simulink model "ssc_hydraulic_lift"  (R2025a)
settings: Solver=ode23t  StartTime=0.0  StopTime=20  MaxStep=0.02  RelTol=1e-3  AbsTol=1e-4  EnableMultiTasking=on
PreLoadFcn:
  | warning('off','Simulink:Commands:LoadMdlParameterizedLink');
PostLoadFcn:
  | warning off sm:compiler:topologyAnalysis:DanglingBlock
  | warning off Simulink:SL_SolverMaskedZC;
  | warning off Simulink:SL_SolverIgnoredZCBracketing;
  | warning off Simulink:Engine:SolverMinStepNonlinearIterWarnForDAE;
  | warning off simscape:compiler:sli:init:SolverNotRecommended
  | warning off Simulink:Engine:UsingDiscreteSolver
  | warning('off','sm:sli:setup:compile:LocalSolverNotSupported')
  | warning off physmod:simscape:compiler:sli:init:SolverNotRecommended
  | warning off sm:sli:visualization:ModelRefNotSupported
  | warning off Simulink:modelReference:ProtectedModelCallbackLostWarning
StartFcn:
  | tic;
StopFcn:
  | Elapsed_Sim_Time = toc;
  | disp(['Elapsed Sim Time = ' num2str(Elapsed_Sim_Time)]);
undefined symbols (not defined in the file): actuator_hs_b, actuator_hs_k, Local, motor_damping, Scissor_Lift_Param, sigbuilder_block, X, Y, Z
libraries: fl_lib x108, sm_lib x41, Scissor_Parts_Lib x24, nesl_utility x6, SimscapeFluids_lib x2, Custom_lib x2, slpidlib x1, fl_ps_legacy_lib x1, ee_lib x1, Motor_Lib x1, sdl_lib x1
(part 2 of 3)

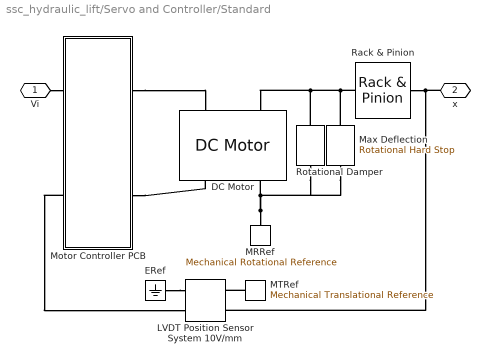
== system ssc_hydraulic_lift/Servo and Controller/Standard ==
  DC Motor : ee_lib/Electromechanical/Brushed Motors/DC Motor  field_option=ee.enum.field_option.pm  Rf=100 Ohm  Lf=1 H  Laf=0.15 H  If0=0 A  parameterization=1  Ra=R Ohm  La=L H  emf_or_torque=1  Kv=Kt V/(rad/s)  Ki=6.876e-4 N*m/A  T_stall=2.4e-4 N*m  w_max=1.91e+4 rpm  w_rated=1.5e+4 rpm  P_rated=0.08 W  V_rated=1.5 V  lam_param=1  i_noload=0 A  V_i_noload=1.5 V  J=J kg*m^2  lam=0 N*m/(rad/s)  speed0=0 rpm  alpha=3.93e-3 1/K  Tmeas=25 degC  thermal_mass=100 J/K  initial_temperature=25 degC
  ERef : fl_lib/Electrical/Electrical Elements/Electrical Reference
  LVDT Position Sensor System 10V/mm : Motor_Lib/Custom/LVDT Position Sensor System 10V//mm  SystemSampleTime=-1  VariantActivationTime=update diagram  EmptyChoice=off  PassThrough=off  PassThroughVariantControl=(default)  EmptyChoiceVariantControl=(default)  AllowFlexibleInterface=on  Latency=0  AutoFrameSizeCalculation=off
  MRRef : fl_lib/Mechanical/Rotational Elements/Mechanical Rotational Reference
  MTRef : fl_lib/Mechanical/Translational Elements/Mechanical Translational Reference
  Max Deflection : fl_lib/Mechanical/Rotational Elements/Rotational Hard Stop  upper_bnd=x_max*1e-3/G rad  lower_bnd=-x_max*1e-3/G rad  model=3  stiff_up=1e+06 N*m/rad  stiff_low=1e+06 N*m/rad  D_up=0.05 N*m/(rad/s)  D_low=0.05 N*m/(rad/s)  transition=0.001 rad  coeff_rest=0.7  w_tol=0.1 rad/s  trq_tol=0.001 N*m  w_specify=off  w_priority=None  w=0 rad/s  w_nominal_specify=off  w_nominal_value=1  w_nominal_unit=rad/s  t_specify=off  t_priority=None  t=0 N*m  t_nominal_specify=off  t_nominal_value=1  t_nominal_unit=N*m  phi_specify=on  phi_priority=High  phi=0 rad  phi_nominal_specify=off  phi_nominal_value=1  phi_nominal_unit=rad  M_specify=off  M_priority=None  M=0
  Motor Controller PCB : Subsystem
  Rack & Pinion : sdl_lib/Gears/Rotational- Translational/Rack & Pinion  param=1  radius=G m  n_teeth=20  x_tooth=5 mm  rack_direction_sign=1  friction_model=1  efficiency=0.8  temperature_TLU=[ 280 300 320 ] K  efficiency_TLU=[ 0.95 0.9 0.85 ]  pwr_thr=0.001 W  mu_visc_P=0 N*m/(rad/s)  mu_visc_R=0 N/(m/s)  thermal_mass=50 J/K  temperature_specify=off  temperature_priority=High  temperature=300 K  temperature_nominal_specify=off  temperature_nominal_value=1  temperature_nominal_unit=K
      settings: InternalSimscapePortConfiguration="{\"Bottom\":[],\"Left\":[{\"id\":\"P\",\"label\":\"P\",\"type\":\"foundation.mechanical.rotational.rotational\"}],\"Right\":[{\"id\":\"R\",\"label\":\"R\",\"type\":\"foundation.mechanical.translational.translational\"}],\"Top\":[]}"
  Rotational Damper : fl_lib/Mechanical/Rotational Elements/Rotational Damper  D=lambda N*m/(rad/s)  w_specify=off  w_priority=None  w=0 rad/s  w_nominal_specify=off  w_nominal_value=1  w_nominal_unit=rad/s  t_specify=off  t_priority=None  t=0 N*m  t_nominal_specify=off  t_nominal_value=1  t_nominal_unit=N*m
  Vi : PMIOPort  Side=Left
  x : PMIOPort  Port=2  Side=Right
  connections:
  Rack & Pinion/RConn1 -- LVDT Position Sensor System 10V/mm/LConn2 -- x/RConn1
  MTRef/LConn1 -- LVDT Position Sensor System 10V/mm/LConn1
  Motor Controller PCB/LConn2 -- LVDT Position Sensor System 10V/mm/RConn2
  ERef/LConn1 -- LVDT Position Sensor System 10V/mm/RConn1
  Motor Controller PCB/RConn2 -- DC Motor/RConn1
  Rack & Pinion/LConn1 -- DC Motor/LConn2 -- Rotational Damper/LConn1 -- Max Deflection/LConn1
  MRRef/LConn1 -- Max Deflection/RConn1 -- Rotational Damper/RConn1 -- DC Motor/RConn2
  Motor Controller PCB/RConn1 -- DC Motor/LConn1
  Vi/RConn1 -- Motor Controller PCB/LConn1

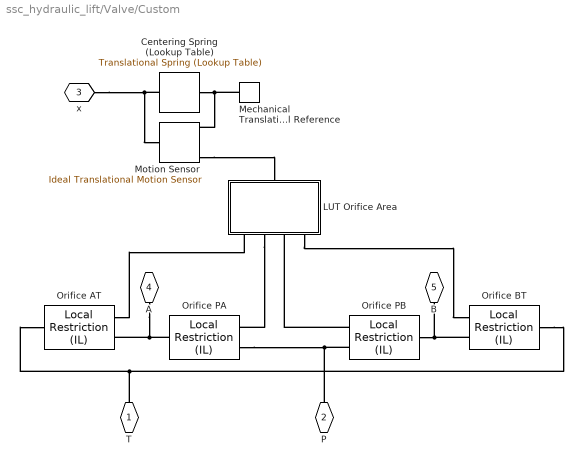
== system ssc_hydraulic_lift/Valve/Custom ==
  Centering Spring (Lookup Table) : Custom_lib/Mechanical/Translational Spring (Lookup Table)  xd=[-1 -0.9 0,0.9 1]*x_max mm  kd=[100,10,10,10,100] N/m  f_specify=off  f_priority=High  f=0 N  f_nominal_specify=off  f_nominal_value=1  f_nominal_unit=N  x_specify=off  x_priority=High  x=0 m  x_nominal_specify=off  x_nominal_value=1  x_nominal_unit=m  v_specify=off  v_priority=High  v=0 m/s  v_nominal_specify=off  v_nominal_value=1  v_nominal_unit=m/s  k_specify=off  k_priority=High  k=0 N/m  k_nominal_specify=off  k_nominal_value=1  k_nominal_unit=N/m
      settings: InternalSimscapePortConfiguration="{\"Bottom\":[],\"Left\":[{\"id\":\"c\",\"label\":\"c\",\"type\":\"foundation.mechanical.translational.translational\"}],\"Right\":[{\"id\":\"r\",\"label\":\"r\",\"type\":\"foundation.mechanical.translational.translational\"}],\"Top\":[]}"
  LUT Orifice Area : Subsystem
  Mechanical Translational Reference : fl_lib/Mechanical/Translational Elements/Mechanical Translational Reference
  Motion Sensor : fl_lib/Mechanical/Mechanical Sensors/Ideal Translational Motion Sensor  reference=foundation.enum.MeasurementReference.difference  acceleration_port=false  velocity_port=true  position_port=true  offset=0 m
  Orifice AT : fl_lib/Isothermal Liquid/Elements/Local Restriction (IL)  restriction_type=foundation.enum.restriction_type.variable  restriction_area=1e-3 m^2  min_area=1e-12 m^2  max_area=1e10 m^2  area=inf m^2  Cd=K_V  Re_c=12  pressure_recovery=false
      settings: LibrarySourceBlock=fl_lib/Isothermal Liquid/Elements/Local Restriction (IL)  InternalSimscapePortConfiguration="{\"Bottom\":[],\"Left\":[{\"id\":\"A\",\"label\":\"A\",\"type\":\"foundation.isothermal_liquid.isothermal_liquid\"},{\"id\":\"AR\",\"label\":\"AR\",\"type\":\"input\"}],\"Right\":[{\"id\":\"B\",\"label\":\"B\",\"type\":\"foundation.isothermal_liquid.isothermal_liquid\"}],\"Top\":[]}"
  Orifice BT : fl_lib/Isothermal Liquid/Elements/Local Restriction (IL)  restriction_type=foundation.enum.restriction_type.variable  restriction_area=1e-3 m^2  min_area=1e-12 m^2  max_area=1e10 m^2  area=inf m^2  Cd=K_V  Re_c=12  pressure_recovery=false
      settings: LibrarySourceBlock=fl_lib/Isothermal Liquid/Elements/Local Restriction (IL)  InternalSimscapePortConfiguration="{\"Bottom\":[],\"Left\":[{\"id\":\"A\",\"label\":\"A\",\"type\":\"foundation.isothermal_liquid.isothermal_liquid\"},{\"id\":\"AR\",\"label\":\"AR\",\"type\":\"input\"}],\"Right\":[{\"id\":\"B\",\"label\":\"B\",\"type\":\"foundation.isothermal_liquid.isothermal_liquid\"}],\"Top\":[]}"
  Orifice PA : fl_lib/Isothermal Liquid/Elements/Local Restriction (IL)  restriction_type=foundation.enum.restriction_type.variable  restriction_area=1e-3 m^2  min_area=1e-12 m^2  max_area=1e10 m^2  area=inf m^2  Cd=K_V  Re_c=12  pressure_recovery=false
      settings: LibrarySourceBlock=fl_lib/Isothermal Liquid/Elements/Local Restriction (IL)  InternalSimscapePortConfiguration="{\"Bottom\":[],\"Left\":[{\"id\":\"A\",\"label\":\"A\",\"type\":\"foundation.isothermal_liquid.isothermal_liquid\"},{\"id\":\"AR\",\"label\":\"AR\",\"type\":\"input\"}],\"Right\":[{\"id\":\"B\",\"label\":\"B\",\"type\":\"foundation.isothermal_liquid.isothermal_liquid\"}],\"Top\":[]}"
  Orifice PB : fl_lib/Isothermal Liquid/Elements/Local Restriction (IL)  restriction_type=foundation.enum.restriction_type.variable  restriction_area=1e-3 m^2  min_area=1e-12 m^2  max_area=1e10 m^2  area=inf m^2  Cd=K_V  Re_c=12  pressure_recovery=false
      settings: LibrarySourceBlock=fl_lib/Isothermal Liquid/Elements/Local Restriction (IL)  InternalSimscapePortConfiguration="{\"Bottom\":[],\"Left\":[{\"id\":\"A\",\"label\":\"A\",\"type\":\"foundation.isothermal_liquid.isothermal_liquid\"},{\"id\":\"AR\",\"label\":\"AR\",\"type\":\"input\"}],\"Right\":[{\"id\":\"B\",\"label\":\"B\",\"type\":\"foundation.isothermal_liquid.isothermal_liquid\"}],\"Top\":[]}"
  T : PMIOPort  Tag=PMCPort  Side=Left
  P : PMIOPort  Tag=PMCPort  Port=2  Side=Left
  x : PMIOPort  Tag=PMCPort  Port=3  Side=Left
  A : PMIOPort  Tag=PMCPort  Port=4  Side=Right
  B : PMIOPort  Tag=PMCPort  Port=5  Side=Right
  connections:
  P/RConn1 -- Orifice PB/LConn1 -- Orifice PA/LConn1
  Mechanical Translational Reference/LConn1 -- Centering Spring (Lookup Table)/RConn1 -- Motion Sensor/RConn1
  x/RConn1 -- Centering Spring (Lookup Table)/LConn1 -- Motion Sensor/LConn1
  Motion Sensor/RConn3 -- LUT Orifice Area/LConn1
  Orifice AT/LConn2 -- LUT Orifice Area/RConn1
  Orifice PB/RConn1 -- Orifice BT/LConn1 -- B/RConn1
  Orifice PB/LConn2 -- LUT Orifice Area/RConn3
  T/RConn1 -- Orifice BT/RConn1 -- Orifice AT/RConn1
  A/RConn1 -- Orifice PA/RConn1 -- Orifice AT/LConn1
  LUT Orifice Area/RConn2 -- Orifice PA/LConn2
  LUT Orifice Area/RConn4 -- Orifice BT/LConn2

== system ssc_hydraulic_lift/Valve/Standard ==
  4-Way Directional Valve : SimscapeFluids_lib/Isothermal Liquid/Valves & Orifices/Directional Control Valves/4-Way 3-Position Directional Valve (IL)  open_orifices_pos=fluids.isothermal_liquid.valves_orifices.directional_control_valves.enum.directional_valve_open_orifices_pos_neg.PA_BT  open_orifices_neu=fluids.isothermal_liquid.valves_orifices.directional_control_valves.enum.directional_valve_open_orifices_neutral.all_closed  open_orifices_neg=fluids.isothermal_liquid.valves_orifices.directional_control_valves.enum.directional_valve_open_orifices_pos_neg.PB_AT  neutral_assert_action=0  area_spec=fluids.isothermal_liquid.valves_orifices.directional_control_valves.enum.directional_valve_area_spec.identical  valve_spec=2  del_S_max=0.0049999 m  area_max=5e-5 m^2  del_S_TLU=[0 x_lap x_max]*1e-3 m  valve_area_TLU=[A_leak*0.1 A_leak A_max] mm^2  del_S_vol_flow_TLU=[0, .00125, .0025, .00375, .005] m  p_diff_TLU=[ -1e+7 -5e+6 -2e+6 2e+6 5e+6 1e+7 ] Pa  vol_flow_TLU=[ -1e-7 -7.0711e-8 -4.4721e-8 4.4721e-8 7.0711e-8 1e-7; -2.0352e-5 -1.4391e-5 -9.1017e-6 9.1017e-6 1.4391e-5 2.0352e-5; -0.0040736 -0.0028805 -0.0018218 0.0018218 0.0028805 0.0040736; -0.011438 -0.0080879 -0.0051152 0.0051152 0.0080879 0.011438; -0.034356 -0.024293 -0.015364 0.015364 0.024293 0.034356 ] m^3/s  p_diff_TLU_const=[-.1, .3, .5, .7] MPa  vol_flow_TLU_const=[-.0009, .0016, .002, .0024] m^3/s  area_const=1e-4 m^2  area_leak=1e-9 m^2  area=inf m^2  Cd=K_V  Re_c=12  smoothing_factor=0  pressure_recovery=false  S_max_PA=x_max mm  del_S_max_PA=0.0049999 m  area_max_PA=0.5e-4 m^2  del_S_TLU_PA=[-x_max -x_lap 0 x_lap x_max 2*x_max]*1e-3 m  valve_area_TLU_PA=[0 0 A_leak 2*A_leak A_max A_max] mm^2  del_S_vol_flow_TLU_PA=[0, .00125, .0025, .00375, .005] m  p_diff_TLU_PA=[-10000000.0, -5000000.0, -2000000.0, 2000000.0, 5000000.0, 10000000.0] Pa  vol_flow_TLU_PA=[-1.0e-7, -7.0711e-8, -4.4721e-8, 4.4721e-8, 7.0711e-8, 1.0e-7; -2.0352e-5, -1.4391e-5, -9.1017e-6, 9.1017e-6, 1.4391e-5, 2.0352e-5; -0.0040736, -0.0028805, -0.0018218, 0.0018218, 0.0028805, 0.0040736; -0.011438, -0.0080879, -0.0051152, 0.0051152, 0.0080879, 0.011438; -0.034356, -0.024293, -0.015364, 0.015364, 0.024293, 0.034356] m^3/s  area_const_PA=1e-4 m^2  p_diff_TLU_const_PA=[-.1, .3, .5, .7] MPa  vol_flow_TLU_const_PA=[-.0009, .0016, .002, .0024] m^3/s  S_max_PB=-x_max mm  del_S_max_PB=0.0049999 m  area_max_PB=0.5e-4 m^2  del_S_TLU_PB=[-x_max -x_lap 0 x_lap x_max 2*x_max]*1e-3 m  valve_area_TLU_PB=[0 0 A_leak 2*A_leak A_max A_max] mm^2  del_S_vol_flow_TLU_PB=[0, .00125, .0025, .00375, .005] m  p_diff_TLU_PB=[-10000000.0, -5000000.0, -2000000.0, 2000000.0, 5000000.0, 10000000.0] Pa  vol_flow_TLU_PB=[-1.0e-7, -7.0711e-8, -4.4721e-8, 4.4721e-8, 7.0711e-8, 1.0e-7; -2.0352e-5, -1.4391e-5, -9.1017e-6, 9.1017e-6, 1.4391e-5, 2.0352e-5; -0.0040736, -0.0028805, -0.0018218, 0.0018218, 0.0028805, 0.0040736; -0.011438, -0.0080879, -0.0051152, 0.0051152, 0.0080879, 0.011438; -0.034356, -0.024293, -0.015364, 0.015364, 0.024293, 0.034356] m^3/s  area_const_PB=1e-4 m^2  p_diff_TLU_const_PB=[-.1, .3, .5, .7] MPa  vol_flow_TLU_const_PB=[-.0009, .0016, .002, .0024] m^3/s  S_max_AB=7.5e-3 m  del_S_max_AB=0.005 m  area_max_AB=1e-4 m^2  del_S_TLU_AB=[0, .00125, .0025, .00375, .005] m  valve_area_TLU_AB=[1e-10, 1e-05, 4e-05, 6e-05, .0001] m^2  del_S_vol_flow_TLU_AB=[0, .00125, .0025, .00375, .005] m  p_diff_TLU_AB=[-.1, .3, .5, .7] MPa  vol_flow_TLU_AB=[-1e-08, 2.2e-08, 2.8e-08, 3.4e-08; -9e-06, .00015, .0002, .00024; -.00036, .00063, .00081, .00096; -.00054, .00094, .0012, .0014; -.00091, .0016, .002, .0024] m^3/s  area_const_AB=1e-4 m^2  p_diff_TLU_const_AB=[-.1, .3, .5, .7] MPa  vol_flow_TLU_const_AB=[-.0009, .0016, .002, .0024] m^3/s  S_max_AT=-x_max mm  del_S_max_AT=0.0049999 m  area_max_AT=0.5e-4 m^2  del_S_TLU_AT=[-x_max -x_lap 0 x_lap x_max 2*x_max]*1e-3 m  valve_area_TLU_AT=[0 0 A_leak 2*A_leak A_max A_max] mm^2  del_S_vol_flow_TLU_AT=[0, .00125, .0025, .00375, .005] m  p_diff_TLU_AT=[-10000000.0, -5000000.0, -2000000.0, 2000000.0, 5000000.0, 10000000.0] Pa  vol_flow_TLU_AT=[-1.0e-7, -7.0711e-8, -4.4721e-8, 4.4721e-8, 7.0711e-8, 1.0e-7; -2.0352e-5, -1.4391e-5, -9.1017e-6, 9.1017e-6, 1.4391e-5, 2.0352e-5; -0.0040736, -0.0028805, -0.0018218, 0.0018218, 0.0028805, 0.0040736; -0.011438, -0.0080879, -0.0051152, 0.0051152, 0.0080879, 0.011438; -0.034356, -0.024293, -0.015364, 0.015364, 0.024293, 0.034356] m^3/s  area_const_AT=1e-4 m^2  p_diff_TLU_const_AT=[-.1, .3, .5, .7] MPa  vol_flow_TLU_const_AT=[-.0009, .0016, .002, .0024] m^3/s  S_max_BT=x_max mm  del_S_max_BT=0.0049999 m  area_max_BT=0.5e-4 m^2  del_S_TLU_BT=[-x_max -x_lap 0 x_lap x_max 2*x_max]*1e-3 m  valve_area_TLU_BT=[0 0 A_leak 2*A_leak A_max A_max] mm^2  del_S_vol_flow_TLU_BT=[0, .00125, .0025, .00375, .005] m  p_diff_TLU_BT=[-10000000.0, -5000000.0, -2000000.0, 2000000.0, 5000000.0, 10000000.0] Pa  vol_flow_TLU_BT=[-1.0e-7, -7.0711e-8, -4.4721e-8, 4.4721e-8, 7.0711e-8, 1.0e-7; -2.0352e-5, -1.4391e-5, -9.1017e-6, 9.1017e-6, 1.4391e-5, 2.0352e-5; -0.0040736, -0.0028805, -0.0018218, 0.0018218, 0.0028805, 0.0040736; -0.011438, -0.0080879, -0.0051152, 0.0051152, 0.0080879, 0.011438; -0.034356, -0.024293, -0.015364, 0.015364, 0.024293, 0.034356] m^3/s  area_const_BT=1e-4 m^2  p_diff_TLU_const_BT=[-.1, .3, .5, .7] MPa  vol_flow_TLU_const_BT=[-.0009, .0016, .002, .0024] m^3/s  S_max_PT=0 m  del_S_max_PT=0.005 m  area_max_PT=1e-4 m^2  del_S_TLU_PT=[0, .00125, .0025, .00375, .005] m  valve_area_TLU_PT=[1e-10, 1e-05, 4e-05, 6e-05, .0001] m^2  del_S_vol_flow_TLU_PT=[0, .00125, .0025, .00375, .005] m  p_diff_TLU_PT=[-.1, .3, .5, .7] MPa  vol_flow_TLU_PT=[-1e-08, 2.2e-08, 2.8e-08, 3.4e-08; -9e-06, .00015, .0002, .00024; -.00036, .00063, .00081, .00096; -.00054, .00094, .0012, .0014; -.00091, .0016, .002, .0024] m^3/s
      settings: LibrarySourceBlock=SimscapeFluids_lib/Isothermal Liquid/Valves & Orifices/Directional Control Valves/4-Way 3-Position Directional Valve (IL)  InternalSimscapePortConfiguration="{\"Bottom\":[{\"id\":\"P\",\"label\":\"P\",\"type\":\"foundation.isothermal_liquid.isothermal_liquid\"},{\"id\":\"T\",\"label\":\"T\",\"type\":\"foundation.isothermal_liquid.isothermal_liquid\"}],\"Left\":[{\"id\":\"S\",\"label\":\"S\",\"type\":\"input\"}],\"Right\":[],\"Top\":[{\"id\":\"A\",\"label\":\"A\",\"type\":\"foundation.isothermal_liquid.isothermal_liquid\"},{\"id\":\"B\",\"label\":\"B\",\"type\":\"foundation.isothermal_liquid.isothermal_liquid\"}]}"
  Centering Spring (Lookup Table) : Custom_lib/Mechanical/Translational Spring (Lookup Table)  xd=[-1 -0.9 0,0.9 1]*x_max mm  kd=[100,10,10,10,100] N/m  f_specify=off  f_priority=High  f=0 N  f_nominal_specify=off  f_nominal_value=1  f_nominal_unit=N  x_specify=off  x_priority=High  x=0 m  x_nominal_specify=off  x_nominal_value=1  x_nominal_unit=m  v_specify=off  v_priority=High  v=0 m/s  v_nominal_specify=off  v_nominal_value=1  v_nominal_unit=m/s  k_specify=off  k_priority=High  k=0 N/m  k_nominal_specify=off  k_nominal_value=1  k_nominal_unit=N/m
      settings: InternalSimscapePortConfiguration="{\"Bottom\":[],\"Left\":[{\"id\":\"c\",\"label\":\"c\",\"type\":\"foundation.mechanical.translational.translational\"}],\"Right\":[{\"id\":\"r\",\"label\":\"r\",\"type\":\"foundation.mechanical.translational.translational\"}],\"Top\":[]}"
  Mechanical Translational Reference : fl_lib/Mechanical/Translational Elements/Mechanical Translational Reference
  Motion Sensor : fl_lib/Mechanical/Mechanical Sensors/Ideal Translational Motion Sensor  reference=foundation.enum.MeasurementReference.difference  acceleration_port=false  velocity_port=true  position_port=true  offset=0 m
  T : PMIOPort  Tag=PMCPort  Side=Left
  P : PMIOPort  Tag=PMCPort  Port=2  Side=Left
  x : PMIOPort  Tag=PMCPort  Port=3  Side=Left
  A : PMIOPort  Tag=PMCPort  Port=4  Side=Right
  B : PMIOPort  Tag=PMCPort  Port=5  Side=Right
  connections:
  Motion Sensor/RConn1 -- Centering Spring (Lookup Table)/RConn1 -- Mechanical Translational Reference/LConn1
  x/RConn1 -- Centering Spring (Lookup Table)/LConn1 -- Motion Sensor/LConn1
  Motion Sensor/RConn3 -- 4-Way Directional Valve/LConn1
  A/RConn1 -- 4-Way Directional Valve/LConn2
  B/RConn1 -- 4-Way Directional Valve/LConn3
  T/RConn1 -- 4-Way Directional Valve/RConn2
  P/RConn1 -- 4-Way Directional Valve/RConn1

== system ssc_hydraulic_lift/Controller/Algorithm/Sensor Gain ==
  Initial Disp : fl_lib/Physical Signals/Sources/PS Constant  constant=Scissor_Lift_Param.Initial_Cyl_Ext mm
  Mid Range 2.5V : fl_lib/Physical Signals/Sources/PS Constant  constant=2.5 V
  PS Add : fl_lib/Physical Signals/Functions/PS Add
  PS Gain : fl_lib/Physical Signals/Functions/PS Gain  gain=Scissor_Lift_Param.Sensor_Gain V/m
  PS Subtract : fl_lib/Physical Signals/Functions/PS Subtract
  Sensor Gain : fl_ps_legacy_lib/Legacy Physical Signals/Functions/PS Gain  gain=Scissor_Lift_Param.Sensor_Gain
  Vout : PMIOPort  Side=Right
  Din : PMIOPort  Port=2  Side=Left
  connections:
  PS Subtract/LConn1 -- Din/RConn1
  PS Gain/LConn1 -- PS Subtract/RConn1
  PS Add/RConn1 -- Vout/RConn1
  PS Subtract/LConn2 -- Initial Disp/RConn1
  PS Gain/RConn1 -- PS Add/LConn1
  PS Add/LConn2 -- Mid Range 2.5V/RConn1

== system ssc_hydraulic_lift/Controller/Algorithm/Voltage Source ==
  V : Inport
  Controlled Voltage Source : fl_lib/Electrical/Electrical Sources/Controlled Voltage Source
  Simulink-PS Converter2 : nesl_utility/Simulink-PS Converter  PhysicalDomain=network_engine_domain  SubClassName=ps_input  LeftPortType=input  RightPortType=output  PseudoPeriodic=off  Frequencies=[]  NoiseDistribution=none  NoiseParameters=[]  Unit=V  AffineConversion=off  FilteringAndDerivatives=filter  SimscapeFilterOrder=1  InputFilterTimeConstant=0.005  UdotUserProvided=1
  + : PMIOPort  Side=Right
  - : PMIOPort  Port=2  Side=Left
  wires:
  V/1 -> Simulink-PS Converter2/1
  connections:
  Controlled Voltage Source/RConn1 -- Simulink-PS Converter2/RConn1
  Controlled Voltage Source/LConn1 -- +/RConn1
  Controlled Voltage Source/RConn2 -- -/RConn1

== system ssc_hydraulic_lift/Controller/Circuit/Sensor Gain ==
  Initial Disp (m) : fl_lib/Physical Signals/Sources/PS Constant  constant=Scissor_Lift_Param.Initial_Cyl_Ext*1e-3 m
  Mid Range 2.5V : fl_lib/Physical Signals/Sources/PS Constant  constant=2.5 V
  PS Add : fl_lib/Physical Signals/Functions/PS Add
  PS Subtract : fl_lib/Physical Signals/Functions/PS Subtract
  Sensor Gain : fl_lib/Physical Signals/Functions/PS Gain  gain=Scissor_Lift_Param.Sensor_Gain V/m
  Vout : PMIOPort  Side=Right
  Din : PMIOPort  Port=2  Side=Left
  connections:
  Mid Range 2.5V/RConn1 -- PS Add/LConn2
  PS Add/LConn1 -- Sensor Gain/RConn1
  Initial Disp (m)/RConn1 -- PS Subtract/LConn2
  Vout/RConn1 -- PS Add/RConn1
  PS Subtract/RConn1 -- Sensor Gain/LConn1
  PS Subtract/LConn1 -- Din/RConn1

== system ssc_hydraulic_lift/Load/Scissor/Actuator ==
  Collar Base : Scissor_Parts_Lib/Collar  collar_length=Scissor_Lift_Param.Actuator.Collar.Length  collar_radius=Scissor_Lift_Param.Actuator.Collar.Radius  cylinder_length=Scissor_Lift_Param.Actuator.Piston_Seat.Length*2  cylinder_radius=Scissor_Lift_Param.Actuator.Piston_Seat.Radius  cylinder_ori=Local +Z  material_density=Scissor_Lift_Param.Actuator.Collar.Density  material_color=Scissor_Lift_Param.Actuator.Collar.Color  material_opacity=Scissor_Lift_Param.Actuator.Collar.Opacity
  Collar Link : Scissor_Parts_Lib/Collar  collar_length=Scissor_Lift_Param.Actuator.Collar.Length  collar_radius=Scissor_Lift_Param.Actuator.Collar.Radius  cylinder_length=Scissor_Lift_Param.Actuator.Piston_Seat.Length*2  cylinder_radius=Scissor_Lift_Param.Actuator.Piston_Seat.Radius  cylinder_ori=Local +Z  material_density=Scissor_Lift_Param.Actuator.Collar.Density  material_color=Scissor_Lift_Param.Actuator.Collar.Color  material_opacity=Scissor_Lift_Param.Actuator.Collar.Opacity
  Piston : Scissor_Parts_Lib/Shaft  L=Scissor_Lift_Param.Actuator.Piston.Length  r=Scissor_Lift_Param.Actuator.Piston.Radius  theta=0  z_ori=Local +Z  Ro=Scissor_Lift_Param.Actuator.Piston.Density  clr=Scissor_Lift_Param.Actuator.Piston.Color  opc=Scissor_Lift_Param.Actuator.Piston.Opacity
  Prismatic Actuator : sm_lib/Joints/Prismatic Joint  JointMode=Normal  CompositeWrenchDir=FollowerOnBase  CompositeWrenchFrame=BaseFrame  SenseConstraintForce=off  SenseConstraintTorque=off  SenseTotalForce=off  SenseTotalTorque=off  PositionTargetSpecify=off  PositionTargetPriority=High  PositionTargetValue=0  PositionTargetValueUnits=m  VelocityTargetSpecify=off  VelocityTargetPriority=High  VelocityTargetValue=0  VelocityTargetValueUnits=m/s  EquilibriumPosition=0  EquilibriumPositionUnits=m  SpringStiffness=0  SpringStiffnessUnits=N/m  DampingCoefficient=Scissor_Lift_Param.Actuator.Damping  DampingCoefficientUnits=N/(m/s)  LowerLimitSpecify=off  LowerLimitBound=-1  LowerLimitBoundUnits=m  LowerLimitStiffness=1e6  LowerLimitStiffnessUnits=N/m  LowerLimitDamping=1e3  LowerLimitDampingUnits=N/(m/s)  LowerLimitTransitionRegionWidth=1e-4  LowerLimitTransitionRegionWidthUnits=m  UpperLimitSpecify=off  UpperLimitBound=1  UpperLimitBoundUnits=m  UpperLimitStiffness=1e6  UpperLimitStiffnessUnits=N/m  UpperLimitDamping=1e3  UpperLimitDampingUnits=N/(m/s)  UpperLimitTransitionRegionWidth=1e-4  UpperLimitTransitionRegionWidthUnits=m  TorqueActuationMode=InputTorque  MotionActuationMode=ComputedMotion  SensePosition=off  SenseVelocity=on  SenseAcceleration=off  SenseTorqueForce=off  SenseLowerLimitTorqueForce=off  SenseUpperLimitTorqueForce=off
  Transform Act Shaft : sm_lib/Frames and Transforms/Rigid Transform  RotationMethod=StandardAxis  FollAlignAxisA=+X  BaseAlignAxisA=+Y  FollAlignAxisB=+Y  BaseAlignAxisB=+Z  RotationStandardAxis=+X  RotationAngle=180  RotationAngleUnits=deg  RotationArbitraryAxis=[0 0 1]  RotationSequenceAxes=FollowerAxes  RotationSequence=XYX  RotationSequenceAngles=[0 0 0]  RotationSequenceAnglesUnits=deg  RotationMatrix=[1 0 0; 0 1 0; 0 0 1]  Quaternion=[1 0 0 0]  TranslationMethod=None  TranslationCartesianOffset=[0 0 0]  TranslationCartesianOffsetUnits=cm  TranslationStandardAxis=-X  TranslationStandardOffset=0  TranslationStandardOffsetUnits=cm  TranslationROffset=0  TranslationROffsetUnits=m  TranslationThetaOffset=0  TranslationThetaOffsetUnits=deg  TranslationZOffset=0  TranslationZOffsetUnits=m
  Translational Simscape Intf : Subsystem
  L : PMIOPort  Side=Right
  B : PMIOPort  Port=2  Side=Left
  C : PMIOPort  Port=3  Side=Left
  R : PMIOPort  Port=4  Side=Right
  connections:
  Collar Base/LConn1 -- B/RConn1
  Transform Act Shaft/RConn1 -- Prismatic Actuator/LConn1
  Prismatic Actuator/LConn2 -- Translational Simscape Intf/LConn1
  Translational Simscape Intf/RConn1 -- Prismatic Actuator/RConn2
  Collar Link/LConn1 -- L/RConn1
  Transform Act Shaft/LConn1 -- Collar Link/RConn1
  Piston/LConn1 -- Collar Base/RConn1
  Piston/RConn1 -- Prismatic Actuator/RConn1
  C/RConn1 -- Translational Simscape Intf/LConn2
  R/RConn1 -- Translational Simscape Intf/RConn2

== system ssc_hydraulic_lift/Load/Scissor/Base ==
  Mechanism Configuration : sm_lib/Utilities/Mechanism Configuration  UniformGravity=Constant  GravityVector=[0 0 -9.81]  GravityVectorUnits=m/s^2  LinearizationDelta=0.001  JointModeTransitionNonlinearIterations=2
  Platform : Subsystem
  Rear Shaft : Subsystem
  Transform Front Roller : sm_lib/Frames and Transforms/Rigid Transform  RotationMethod=StandardAxis  FollAlignAxisA=+X  BaseAlignAxisA=+Y  FollAlignAxisB=+Y  BaseAlignAxisB=+Z  RotationStandardAxis=+Y  RotationAngle=90  RotationAngleUnits=deg  RotationArbitraryAxis=[0 0 1]  RotationSequenceAxes=FollowerAxes  RotationSequence=XYX  RotationSequenceAngles=[0 0 0]  RotationSequenceAnglesUnits=deg  RotationMatrix=[1 0 0; 0 1 0; 0 0 1]  Quaternion=[1 0 0 0]  TranslationMethod=Cartesian  TranslationCartesianOffset=[-Scissor_Lift_Param.Link.Length -Scissor_Lift_Param.Base_Block.Height/2 0]  TranslationCartesianOffsetUnits=cm  TranslationStandardAxis=-X  TranslationStandardOffset=0  TranslationStandardOffsetUnits=cm  TranslationROffset=0  TranslationROffsetUnits=m  TranslationThetaOffset=0  TranslationThetaOffsetUnits=deg  TranslationZOffset=0  TranslationZOffsetUnits=m
  World Frame : sm_lib/Frames and Transforms/World Frame
  Front : PMIOPort  Side=Right
  Rear : PMIOPort  Port=2  Side=Right
  connections:
  Front/RConn1 -- Transform Front Roller/RConn1
  Rear/RConn1 -- Transform Front Roller/LConn1 -- Rear Shaft/RConn1
  World Frame/RConn1 -- Mechanism Configuration/RConn1 -- Platform/LConn1
  Platform/RConn1 -- Rear Shaft/LConn1

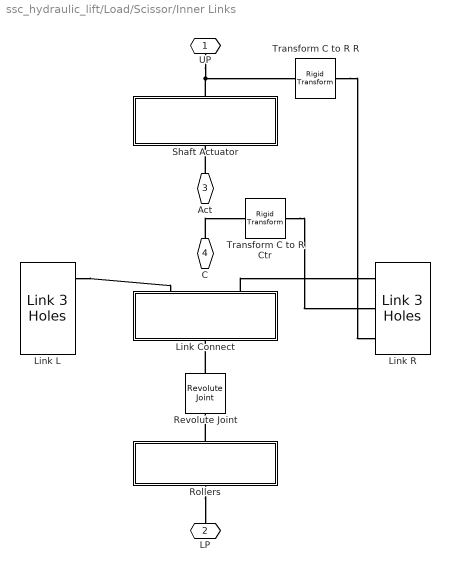
== system ssc_hydraulic_lift/Load/Scissor/Inner Links ==
  Link Connect : Subsystem
  Link L : Scissor_Parts_Lib/Link 3 Holes  L=Scissor_Lift_Param.Link.Length  W=Scissor_Lift_Param.Link.Width  T=Scissor_Lift_Param.Link.Thickness  r=Scissor_Lift_Param.Link.Hole_Radius  rho=Scissor_Lift_Param.Link.Density  clr_string=Yellow  opc=Scissor_Lift_Param.Link.Opacity
  Link R : Scissor_Parts_Lib/Link 3 Holes  L=Scissor_Lift_Param.Link.Length  W=Scissor_Lift_Param.Link.Width  T=Scissor_Lift_Param.Link.Thickness  r=Scissor_Lift_Param.Link.Hole_Radius  rho=Scissor_Lift_Param.Link.Density  clr_string=Yellow  opc=Scissor_Lift_Param.Link.Opacity
  Revolute Joint : sm_lib/Joints/Revolute Joint  JointMode=Normal  CompositeWrenchDir=FollowerOnBase  CompositeWrenchFrame=BaseFrame  SenseConstraintForce=off  SenseConstraintTorque=off  SenseTotalForce=off  SenseTotalTorque=off  PositionTargetSpecify=off  PositionTargetPriority=High  PositionTargetValue=0  PositionTargetValueUnits=deg  VelocityTargetSpecify=off  VelocityTargetPriority=High  VelocityTargetValue=0  VelocityTargetValueUnits=deg/s  EquilibriumPosition=0  EquilibriumPositionUnits=deg  SpringStiffness=0  SpringStiffnessUnits=N*m/deg  DampingCoefficient=0  DampingCoefficientUnits=N*m/(deg/s)  LowerLimitSpecify=off  LowerLimitBound=-90  LowerLimitBoundUnits=deg  LowerLimitStiffness=1e4  LowerLimitStiffnessUnits=N*m/deg  LowerLimitDamping=10  LowerLimitDampingUnits=N*m/(deg/s)  LowerLimitTransitionRegionWidth=0.1  LowerLimitTransitionRegionWidthUnits=deg  UpperLimitSpecify=off  UpperLimitBound=90  UpperLimitBoundUnits=deg  UpperLimitStiffness=1e4  UpperLimitStiffnessUnits=N*m/deg  UpperLimitDamping=10  UpperLimitDampingUnits=N*m/(deg/s)  UpperLimitTransitionRegionWidth=0.1  UpperLimitTransitionRegionWidthUnits=deg  TorqueActuationMode=NoTorque  MotionActuationMode=ComputedMotion  SensePosition=off  SenseVelocity=off  SenseAcceleration=off  SenseTorqueForce=off  SenseLowerLimitTorqueForce=off  SenseUpperLimitTorqueForce=off
  Rollers : Subsystem
  Shaft Actuator : Subsystem
  Transform C to R Ctr : sm_lib/Frames and Transforms/Rigid Transform  RotationMethod=None  FollAlignAxisA=+X  BaseAlignAxisA=+Y  FollAlignAxisB=+Y  BaseAlignAxisB=+Z  RotationStandardAxis=+X  RotationAngle=90  RotationAngleUnits=deg  RotationArbitraryAxis=[0 0 1]  RotationSequenceAxes=FollowerAxes  RotationSequence=XYX  RotationSequenceAngles=[0 0 0]  RotationSequenceAnglesUnits=deg  RotationMatrix=[1 0 0; 0 1 0; 0 0 1]  Quaternion=[1 0 0 0]  TranslationMethod=StandardAxis  TranslationCartesianOffset=[0 0 0]  TranslationCartesianOffsetUnits=cm  TranslationStandardAxis=-Z  TranslationStandardOffset=Scissor_Lift_Param.Link_Separation.Inner_Inner/2  TranslationStandardOffsetUnits=cm  TranslationROffset=0  TranslationROffsetUnits=m  TranslationThetaOffset=0  TranslationThetaOffsetUnits=deg  TranslationZOffset=0  TranslationZOffsetUnits=m
  Transform C to R R : sm_lib/Frames and Transforms/Rigid Transform  RotationMethod=None  FollAlignAxisA=+X  BaseAlignAxisA=+Y  FollAlignAxisB=+Y  BaseAlignAxisB=+Z  RotationStandardAxis=+X  RotationAngle=90  RotationAngleUnits=deg  RotationArbitraryAxis=[0 0 1]  RotationSequenceAxes=FollowerAxes  RotationSequence=XYX  RotationSequenceAngles=[0 0 0]  RotationSequenceAnglesUnits=deg  RotationMatrix=[1 0 0; 0 1 0; 0 0 1]  Quaternion=[1 0 0 0]  TranslationMethod=StandardAxis  TranslationCartesianOffset=[0 0 0]  TranslationCartesianOffsetUnits=cm  TranslationStandardAxis=-Z  TranslationStandardOffset=Scissor_Lift_Param.Link_Separation.Inner_Inner/2  TranslationStandardOffsetUnits=cm  TranslationROffset=0  TranslationROffsetUnits=m  TranslationThetaOffset=0  TranslationThetaOffsetUnits=deg  TranslationZOffset=0  TranslationZOffsetUnits=m
  UP : PMIOPort  Side=Left
  LP : PMIOPort  Port=2  Side=Right
  Act : PMIOPort  Port=3  Side=Right
  C : PMIOPort  Port=4  Side=Left
  connections:
  Transform C to R R/RConn1 -- Link R/RConn3
  UP/RConn1 -- Shaft Actuator/LConn1 -- Transform C to R R/LConn1
  Transform C to R Ctr/RConn1 -- Link R/RConn2
  C/RConn1 -- Transform C to R Ctr/LConn1
  Rollers/RConn1 -- Revolute Joint/RConn1
  Rollers/LConn1 -- LP/RConn1
  Act/RConn1 -- Shaft Actuator/RConn1
  Link Connect/RConn2 -- Link R/RConn1
  Link L/RConn1 -- Link Connect/RConn1
  Revolute Joint/LConn1 -- Link Connect/LConn1

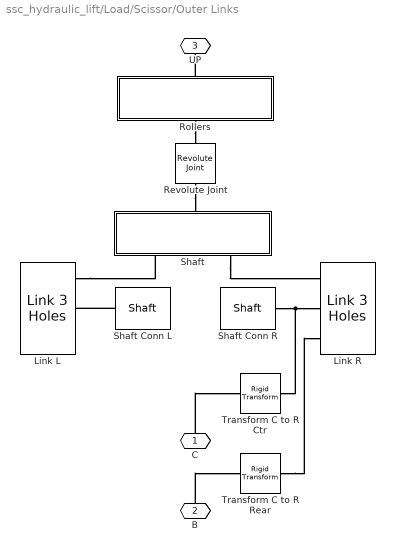
== system ssc_hydraulic_lift/Load/Scissor/Outer Links ==
  Link L : Scissor_Parts_Lib/Link 3 Holes  L=Scissor_Lift_Param.Link.Length  W=Scissor_Lift_Param.Link.Width  T=Scissor_Lift_Param.Link.Thickness  r=Scissor_Lift_Param.Link.Hole_Radius  rho=Scissor_Lift_Param.Link.Density  clr_string=Red  opc=Scissor_Lift_Param.Link.Opacity
  Link R : Scissor_Parts_Lib/Link 3 Holes  L=Scissor_Lift_Param.Link.Length  W=Scissor_Lift_Param.Link.Width  T=Scissor_Lift_Param.Link.Thickness  r=Scissor_Lift_Param.Link.Hole_Radius  rho=Scissor_Lift_Param.Link.Density  clr_string=Red  opc=Scissor_Lift_Param.Link.Opacity
  Revolute Joint : sm_lib/Joints/Revolute Joint  JointMode=Normal  CompositeWrenchDir=FollowerOnBase  CompositeWrenchFrame=BaseFrame  SenseConstraintForce=off  SenseConstraintTorque=off  SenseTotalForce=off  SenseTotalTorque=off  PositionTargetSpecify=off  PositionTargetPriority=High  PositionTargetValue=0  PositionTargetValueUnits=deg  VelocityTargetSpecify=off  VelocityTargetPriority=High  VelocityTargetValue=0  VelocityTargetValueUnits=deg/s  EquilibriumPosition=0  EquilibriumPositionUnits=deg  SpringStiffness=0  SpringStiffnessUnits=N*m/deg  DampingCoefficient=0  DampingCoefficientUnits=N*m/(deg/s)  LowerLimitSpecify=off  LowerLimitBound=-90  LowerLimitBoundUnits=deg  LowerLimitStiffness=1e4  LowerLimitStiffnessUnits=N*m/deg  LowerLimitDamping=10  LowerLimitDampingUnits=N*m/(deg/s)  LowerLimitTransitionRegionWidth=0.1  LowerLimitTransitionRegionWidthUnits=deg  UpperLimitSpecify=off  UpperLimitBound=90  UpperLimitBoundUnits=deg  UpperLimitStiffness=1e4  UpperLimitStiffnessUnits=N*m/deg  UpperLimitDamping=10  UpperLimitDampingUnits=N*m/(deg/s)  UpperLimitTransitionRegionWidth=0.1  UpperLimitTransitionRegionWidthUnits=deg  TorqueActuationMode=NoTorque  MotionActuationMode=ComputedMotion  SensePosition=off  SenseVelocity=off  SenseAcceleration=off  SenseTorqueForce=off  SenseLowerLimitTorqueForce=off  SenseUpperLimitTorqueForce=off
  Rollers : Subsystem
  Shaft : Subsystem
  Shaft Conn L : Scissor_Parts_Lib/Shaft  L=Scissor_Lift_Param.Conn_Shaft.Length  r=Scissor_Lift_Param.Trans_Shaft.Radius  theta=0  z_ori=Local -Z  Ro=Scissor_Lift_Param.Trans_Shaft.Density  clr=Scissor_Lift_Param.Conn_Shaft.Color  opc=Scissor_Lift_Param.Trans_Shaft.Opacity
  Shaft Conn R : Scissor_Parts_Lib/Shaft  L=Scissor_Lift_Param.Conn_Shaft.Length  r=Scissor_Lift_Param.Trans_Shaft.Radius  theta=0  z_ori=Local +Z  Ro=Scissor_Lift_Param.Trans_Shaft.Density  clr=Scissor_Lift_Param.Conn_Shaft.Color  opc=Scissor_Lift_Param.Trans_Shaft.Opacity
  Transform C to R Ctr : sm_lib/Frames and Transforms/Rigid Transform  RotationMethod=None  FollAlignAxisA=+X  BaseAlignAxisA=+Y  FollAlignAxisB=+Y  BaseAlignAxisB=+Z  RotationStandardAxis=+X  RotationAngle=90  RotationAngleUnits=deg  RotationArbitraryAxis=[0 0 1]  RotationSequenceAxes=FollowerAxes  RotationSequence=XYX  RotationSequenceAngles=[0 0 0]  RotationSequenceAnglesUnits=deg  RotationMatrix=[1 0 0; 0 1 0; 0 0 1]  Quaternion=[1 0 0 0]  TranslationMethod=StandardAxis  TranslationCartesianOffset=[0 0 0]  TranslationCartesianOffsetUnits=cm  TranslationStandardAxis=-Z  TranslationStandardOffset=Scissor_Lift_Param.Link_Separation.Outer_Outer/2  TranslationStandardOffsetUnits=cm  TranslationROffset=0  TranslationROffsetUnits=m  TranslationThetaOffset=0  TranslationThetaOffsetUnits=deg  TranslationZOffset=0  TranslationZOffsetUnits=m
  "Transform C to R Rear " : sm_lib/Frames and Transforms/Rigid Transform  RotationMethod=None  FollAlignAxisA=+X  BaseAlignAxisA=+Y  FollAlignAxisB=+Y  BaseAlignAxisB=+Z  RotationStandardAxis=+X  RotationAngle=90  RotationAngleUnits=deg  RotationArbitraryAxis=[0 0 1]  RotationSequenceAxes=FollowerAxes  RotationSequence=XYX  RotationSequenceAngles=[0 0 0]  RotationSequenceAnglesUnits=deg  RotationMatrix=[1 0 0; 0 1 0; 0 0 1]  Quaternion=[1 0 0 0]  TranslationMethod=StandardAxis  TranslationCartesianOffset=[0 0 0]  TranslationCartesianOffsetUnits=cm  TranslationStandardAxis=-Z  TranslationStandardOffset=Scissor_Lift_Param.Link_Separation.Outer_Outer/2  TranslationStandardOffsetUnits=cm  TranslationROffset=0  TranslationROffsetUnits=m  TranslationThetaOffset=0  TranslationThetaOffsetUnits=deg  TranslationZOffset=0  TranslationZOffsetUnits=m
  C : PMIOPort  Side=Right
  B : PMIOPort  Port=2  Side=Left
  UP : PMIOPort  Port=3  Side=Right
  connections:
  B/RConn1 -- "Transform C to R Rear "/LConn1
  "Transform C to R Rear "/RConn1 -- Link R/RConn3
  Transform C to R Ctr/RConn1 -- Link R/RConn2 -- Shaft Conn R/LConn1
  C/RConn1 -- Transform C to R Ctr/LConn1
  Rollers/RConn1 -- UP/RConn1
  Rollers/LConn1 -- Revolute Joint/RConn1
  Revolute Joint/LConn1 -- Shaft/LConn1
  Link L/RConn1 -- Shaft/RConn1
  Shaft/RConn2 -- Link R/RConn1
  Shaft Conn L/LConn1 -- Link L/RConn2

== system ssc_hydraulic_lift/Load/Scissor/Upper Platform ==
  Blocks : Subsystem
  Load : Scissor_Parts_Lib/Block  L=Scissor_Lift_Param.Load.Length  W=Scissor_Lift_Param.Load.Width  H=Scissor_Lift_Param.Load.Height  z_ori=Local +Z  rho=Scissor_Lift_Param.Load.Density  clr=Scissor_Lift_Param.Load.Color  opc=Scissor_Lift_Param.Load.Opacity
  Platform : Scissor_Parts_Lib/Block  L=Scissor_Lift_Param.Upper_Platform.Height  W=Scissor_Lift_Param.Upper_Platform.Width  H=Scissor_Lift_Param.Upper_Platform.Length  z_ori=Local +Z  rho=Scissor_Lift_Param.Upper_Platform.Density  clr=Scissor_Lift_Param.Upper_Platform.Color  opc=Scissor_Lift_Param.Upper_Platform.Opacity
  Transform CG to R : sm_lib/Frames and Transforms/Rigid Transform  RotationMethod=StandardAxis  FollAlignAxisA=+X  BaseAlignAxisA=+Y  FollAlignAxisB=+Y  BaseAlignAxisB=+Z  RotationStandardAxis=+Y  RotationAngle=-90  RotationAngleUnits=deg  RotationArbitraryAxis=[0 0 1]  RotationSequenceAxes=FollowerAxes  RotationSequence=XYX  RotationSequenceAngles=[0 0 0]  RotationSequenceAnglesUnits=deg  RotationMatrix=[1 0 0; 0 1 0; 0 0 1]  Quaternion=[1 0 0 0]  TranslationMethod=Cartesian  TranslationCartesianOffset=[0 0 Scissor_Lift_Param.Link.Length/2]  TranslationCartesianOffsetUnits=cm  TranslationStandardAxis=+Y  TranslationStandardOffset=0  TranslationStandardOffsetUnits=cm  TranslationROffset=0  TranslationROffsetUnits=m  TranslationThetaOffset=0  TranslationThetaOffsetUnits=deg  TranslationZOffset=0  TranslationZOffsetUnits=m
  Transform F to CG : sm_lib/Frames and Transforms/Rigid Transform  RotationMethod=None  FollAlignAxisA=+X  BaseAlignAxisA=+Y  FollAlignAxisB=+Y  BaseAlignAxisB=+Z  RotationStandardAxis=+Z  RotationAngle=0  RotationAngleUnits=deg  RotationArbitraryAxis=[0 0 1]  RotationSequenceAxes=FollowerAxes  RotationSequence=XYX  RotationSequenceAngles=[0 0 0]  RotationSequenceAnglesUnits=deg  RotationMatrix=[1 0 0; 0 1 0; 0 0 1]  Quaternion=[1 0 0 0]  TranslationMethod=Cartesian  TranslationCartesianOffset=[0 0 Scissor_Lift_Param.Link.Length/2]  TranslationCartesianOffsetUnits=cm  TranslationStandardAxis=+Y  TranslationStandardOffset=0  TranslationStandardOffsetUnits=cm  TranslationROffset=0  TranslationROffsetUnits=m  TranslationThetaOffset=0  TranslationThetaOffsetUnits=deg  TranslationZOffset=0  TranslationZOffsetUnits=m
  Transform Orient Platform : sm_lib/Frames and Transforms/Rigid Transform  RotationMethod=StandardAxis  FollAlignAxisA=+X  BaseAlignAxisA=+Y  FollAlignAxisB=+Y  BaseAlignAxisB=+Z  RotationStandardAxis=-X  RotationAngle=90  RotationAngleUnits=deg  RotationArbitraryAxis=[0 0 1]  RotationSequenceAxes=FollowerAxes  RotationSequence=XYX  RotationSequenceAngles=[0 0 0]  RotationSequenceAnglesUnits=deg  RotationMatrix=[1 0 0; 0 1 0; 0 0 1]  Quaternion=[1 0 0 0]  TranslationMethod=None  TranslationCartesianOffset=[0 0 0]  TranslationCartesianOffsetUnits=cm  TranslationStandardAxis=+Y  TranslationStandardOffset=0  TranslationStandardOffsetUnits=cm  TranslationROffset=0  TranslationROffsetUnits=m  TranslationThetaOffset=0  TranslationThetaOffsetUnits=deg  TranslationZOffset=0  TranslationZOffsetUnits=m
  Rear : PMIOPort  Side=Left
  Front : PMIOPort  Port=2  Side=Left
  connections:
  Load/LConn1 -- Platform/RConn1
  Platform/LConn1 -- Transform Orient Platform/RConn1
  Transform CG to R/LConn1 -- Transform Orient Platform/LConn1 -- Transform F to CG/RConn1
  Transform F to CG/LConn1 -- Front/RConn1
  Transform CG to R/RConn1 -- Blocks/RConn1
  Rear/RConn1 -- Blocks/LConn1

== system ssc_hydraulic_lift/Servo and Controller/Custom/LVDT Position Sensor System 10V//mm ==
  10V/mm : fl_lib/Physical Signals/Functions/PS Gain  gain=10 V/mm
  Controlled Voltage Source : fl_lib/Electrical/Electrical Sources/Controlled Voltage Source
  Motion Sensor : fl_lib/Mechanical/Mechanical Sensors/Ideal Translational Motion Sensor  reference=foundation.enum.MeasurementReference.difference  acceleration_port=false  velocity_port=true  position_port=true  offset=0 m
  - : PMIOPort  Side=Right
  + : PMIOPort  Port=2  Side=Right
  C : PMIOPort  Port=3  Side=Left
  R : PMIOPort  Port=4  Side=Left
  connections:
  +/RConn1 -- Controlled Voltage Source/LConn1
  -/RConn1 -- Controlled Voltage Source/RConn2
  R/RConn1 -- Motion Sensor/LConn1
  10V/mm/RConn1 -- Controlled Voltage Source/RConn1
  C/RConn1 -- Motion Sensor/RConn1
  Motion Sensor/RConn3 -- 10V/mm/LConn1

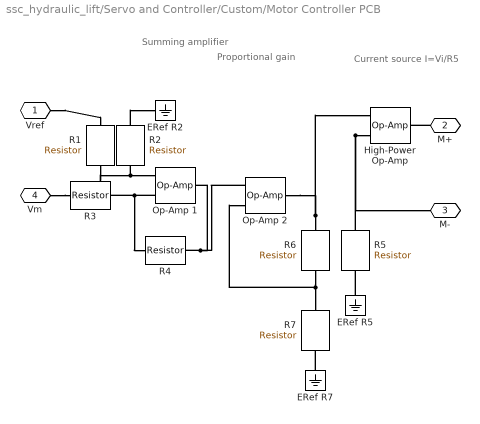
== system ssc_hydraulic_lift/Servo and Controller/Custom/Motor Controller PCB ==
  note: Proportional gain
  note: Summing
      | amplifier
  note: Current source
      | I=Vi/R5
  ERef R2 : fl_lib/Electrical/Electrical Elements/Electrical Reference
  ERef R5 : fl_lib/Electrical/Electrical Elements/Electrical Reference
  ERef R7 : fl_lib/Electrical/Electrical Elements/Electrical Reference
  High-Power Op-Amp : fl_lib/Electrical/Electrical Elements/Op-Amp  outI_specify=off  outI_priority=High  outI=0 A  outI_nominal_specify=off  outI_nominal_value=1  outI_nominal_unit=A
  Op-Amp 1 : fl_lib/Electrical/Electrical Elements/Op-Amp  outI_specify=off  outI_priority=None  outI=0 A  outI_nominal_specify=off  outI_nominal_value=1  outI_nominal_unit=A
  Op-Amp 2 : fl_lib/Electrical/Electrical Elements/Op-Amp  outI_specify=off  outI_priority=None  outI=0 A  outI_nominal_specify=off  outI_nominal_value=1  outI_nominal_unit=A
  R1 : fl_lib/Electrical/Electrical Elements/Resistor  R=R_controller(1) Ohm  i_specify=off  i_priority=High  i=0 A  i_nominal_specify=off  i_nominal_value=1  i_nominal_unit=A  v_specify=off  v_priority=High  v=0 V  v_nominal_specify=off  v_nominal_value=1  v_nominal_unit=V
  R2 : fl_lib/Electrical/Electrical Elements/Resistor  R=R_controller(2) Ohm  i_specify=off  i_priority=None  i=0 A  i_nominal_specify=off  i_nominal_value=1  i_nominal_unit=A  v_specify=off  v_priority=None  v=0 V  v_nominal_specify=off  v_nominal_value=1  v_nominal_unit=V
  R3 : fl_lib/Electrical/Electrical Elements/Resistor  R=R_controller(3) Ohm  i_specify=off  i_priority=High  i=0 A  i_nominal_specify=off  i_nominal_value=1  i_nominal_unit=A  v_specify=off  v_priority=High  v=0 V  v_nominal_specify=off  v_nominal_value=1  v_nominal_unit=V
  R4 : fl_lib/Electrical/Electrical Elements/Resistor  R=R_controller(4) Ohm  i_specify=off  i_priority=None  i=0 A  i_nominal_specify=off  i_nominal_value=1  i_nominal_unit=A  v_specify=off  v_priority=None  v=0 V  v_nominal_specify=off  v_nominal_value=1  v_nominal_unit=V
  R5 : fl_lib/Electrical/Electrical Elements/Resistor  R=R_controller(5) Ohm  i_specify=off  i_priority=High  i=0 A  i_nominal_specify=off  i_nominal_value=1  i_nominal_unit=A  v_specify=off  v_priority=High  v=0 V  v_nominal_specify=off  v_nominal_value=1  v_nominal_unit=V
  R6 : fl_lib/Electrical/Electrical Elements/Resistor  R=R_controller(6) Ohm  i_specify=off  i_priority=None  i=0 A  i_nominal_specify=off  i_nominal_value=1  i_nominal_unit=A  v_specify=off  v_priority=None  v=0 V  v_nominal_specify=off  v_nominal_value=1  v_nominal_unit=V
  R7 : fl_lib/Electrical/Electrical Elements/Resistor  R=R_controller(7) Ohm  i_specify=off  i_priority=None  i=0 A  i_nominal_specify=off  i_nominal_value=1  i_nominal_unit=A  v_specify=off  v_priority=None  v=0 V  v_nominal_specify=off  v_nominal_value=1  v_nominal_unit=V
  Vref : PMIOPort  Side=Left
  M+ : PMIOPort  Port=2  Side=Right
  M- : PMIOPort  Port=3  Side=Right
  Vm : PMIOPort  Port=4  Side=Left
  connections:
  High-Power Op-Amp/LConn2 -- M-/RConn1 -- R5/LConn1
  Vm/RConn1 -- R3/LConn1
  M+/RConn1 -- High-Power Op-Amp/RConn1
  Vref/RConn1 -- R1/LConn1
  R6/RConn1 -- R7/LConn1 -- Op-Amp 2/LConn2
  R4/RConn1 -- Op-Amp 1/RConn1 -- Op-Amp 2/LConn1
  Op-Amp 1/LConn2 -- R4/LConn1 -- R3/RConn1
  R1/RConn1 -- Op-Amp 1/LConn1 -- R2/LConn1
  R6/LConn1 -- Op-Amp 2/RConn1 -- High-Power Op-Amp/LConn1
  ERef R5/LConn1 -- R5/RConn1
  R2/RConn1 -- ERef R2/LConn1
  ERef R7/LConn1 -- R7/RConn1

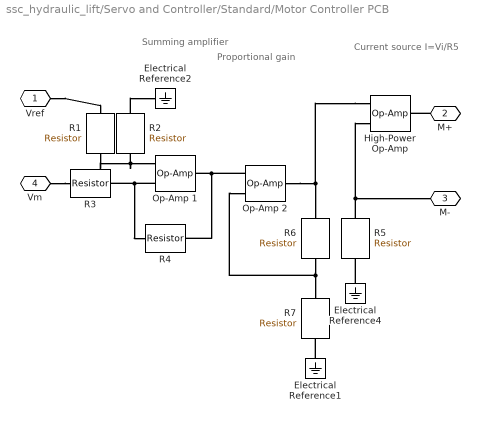
== system ssc_hydraulic_lift/Servo and Controller/Standard/Motor Controller PCB ==
  note: Current source
      | I=Vi/R5
  note: Summing
      | amplifier
  note: Proportional gain
  Electrical Reference1 : fl_lib/Electrical/Electrical Elements/Electrical Reference
  Electrical Reference2 : fl_lib/Electrical/Electrical Elements/Electrical Reference
  Electrical Reference4 : fl_lib/Electrical/Electrical Elements/Electrical Reference
  High-Power Op-Amp : fl_lib/Electrical/Electrical Elements/Op-Amp  outI_specify=off  outI_priority=High  outI=0 A  outI_nominal_specify=off  outI_nominal_value=1  outI_nominal_unit=A
  Op-Amp 1 : fl_lib/Electrical/Electrical Elements/Op-Amp  outI_specify=off  outI_priority=None  outI=0 A  outI_nominal_specify=off  outI_nominal_value=1  outI_nominal_unit=A
  Op-Amp 2 : fl_lib/Electrical/Electrical Elements/Op-Amp  outI_specify=off  outI_priority=None  outI=0 A  outI_nominal_specify=off  outI_nominal_value=1  outI_nominal_unit=A
  R1 : fl_lib/Electrical/Electrical Elements/Resistor  R=R_controller(1) Ohm  i_specify=off  i_priority=High  i=0 A  i_nominal_specify=off  i_nominal_value=1  i_nominal_unit=A  v_specify=off  v_priority=High  v=0 V  v_nominal_specify=off  v_nominal_value=1  v_nominal_unit=V
  R2 : fl_lib/Electrical/Electrical Elements/Resistor  R=R_controller(2) Ohm  i_specify=off  i_priority=None  i=0 A  i_nominal_specify=off  i_nominal_value=1  i_nominal_unit=A  v_specify=off  v_priority=None  v=0 V  v_nominal_specify=off  v_nominal_value=1  v_nominal_unit=V
  R3 : fl_lib/Electrical/Electrical Elements/Resistor  R=R_controller(3) Ohm  i_specify=off  i_priority=High  i=0 A  i_nominal_specify=off  i_nominal_value=1  i_nominal_unit=A  v_specify=off  v_priority=High  v=0 V  v_nominal_specify=off  v_nominal_value=1  v_nominal_unit=V
  R4 : fl_lib/Electrical/Electrical Elements/Resistor  R=R_controller(4) Ohm  i_specify=off  i_priority=None  i=0 A  i_nominal_specify=off  i_nominal_value=1  i_nominal_unit=A  v_specify=off  v_priority=None  v=0 V  v_nominal_specify=off  v_nominal_value=1  v_nominal_unit=V
  R5 : fl_lib/Electrical/Electrical Elements/Resistor  R=R_controller(5) Ohm  i_specify=off  i_priority=High  i=0 A  i_nominal_specify=off  i_nominal_value=1  i_nominal_unit=A  v_specify=off  v_priority=High  v=0 V  v_nominal_specify=off  v_nominal_value=1  v_nominal_unit=V
  R6 : fl_lib/Electrical/Electrical Elements/Resistor  R=R_controller(6) Ohm  i_specify=off  i_priority=None  i=0 A  i_nominal_specify=off  i_nominal_value=1  i_nominal_unit=A  v_specify=off  v_priority=None  v=0 V  v_nominal_specify=off  v_nominal_value=1  v_nominal_unit=V
  R7 : fl_lib/Electrical/Electrical Elements/Resistor  R=R_controller(7) Ohm  i_specify=off  i_priority=None  i=0 A  i_nominal_specify=off  i_nominal_value=1  i_nominal_unit=A  v_specify=off  v_priority=None  v=0 V  v_nominal_specify=off  v_nominal_value=1  v_nominal_unit=V
  Vref : PMIOPort  Side=Left
  M+ : PMIOPort  Port=2  Side=Right
  M- : PMIOPort  Port=3  Side=Right
  Vm : PMIOPort  Port=4  Side=Left
  connections:
  High-Power Op-Amp/LConn2 -- M-/RConn1 -- R5/LConn1
  Electrical Reference1/LConn1 -- R7/RConn1
  R2/RConn1 -- Electrical Reference2/LConn1
  Electrical Reference4/LConn1 -- R5/RConn1
  High-Power Op-Amp/LConn1 -- Op-Amp 2/RConn1 -- R6/LConn1
  R2/LConn1 -- Op-Amp 1/LConn1 -- R1/RConn1
  R3/RConn1 -- R4/LConn1 -- Op-Amp 1/LConn2
  Op-Amp 2/LConn1 -- Op-Amp 1/RConn1 -- R4/RConn1
  Op-Amp 2/LConn2 -- R7/LConn1 -- R6/RConn1
  Vref/RConn1 -- R1/LConn1
  M+/RConn1 -- High-Power Op-Amp/RConn1
  Vm/RConn1 -- R3/LConn1

== system ssc_hydraulic_lift/Valve/Custom/LUT Orifice Area ==
  Area A-T : fl_lib/Physical Signals/Lookup Tables/PS Lookup Table (1D)  x=[-x_max -x_lap 0 x_lap x_max 2*x_max]*1e-3 m  f=[0 0 A_leak 2*A_leak A_max A_max]*1e-6 m^2  interp_method=simscape.enum.interpolation.linear  extrap_method=simscape.enum.extrapolation.linear
  Area B-T : fl_lib/Physical Signals/Lookup Tables/PS Lookup Table (1D)  x=[-x_max -x_lap 0 x_lap x_max 2*x_max]*1e-3 m  f=[0 0 A_leak 2*A_leak A_max A_max]*1e-6 m^2  interp_method=simscape.enum.interpolation.linear  extrap_method=simscape.enum.extrapolation.linear
  Area P-A : fl_lib/Physical Signals/Lookup Tables/PS Lookup Table (1D)  x=[-x_max -x_lap 0 x_lap x_max 2*x_max]*1e-3 m  f=[0 0 A_leak 2*A_leak A_max A_max]*1e-6 m^2  interp_method=simscape.enum.interpolation.linear  extrap_method=simscape.enum.extrapolation.linear
  Area P-B : fl_lib/Physical Signals/Lookup Tables/PS Lookup Table (1D)  x=[-x_max -x_lap 0 x_lap x_max 2*x_max]*1e-3 m  f=[0 0 A_leak 2*A_leak A_max A_max]*1e-6 m^2  interp_method=simscape.enum.interpolation.linear  extrap_method=simscape.enum.extrapolation.linear
  Reverse Direction : fl_lib/Physical Signals/Functions/PS Gain  gain=-1
  Disp : PMIOPort  Side=Left
  A-T : PMIOPort  Port=2  Side=Right
  P-A : PMIOPort  Port=3  Side=Right
  B-P : PMIOPort  Port=4  Side=Right
  B-T : PMIOPort  Port=5  Side=Right
  connections:
  Area P-A/RConn1 -- P-A/RConn1
  Area P-A/LConn1 -- Area B-T/LConn1 -- Reverse Direction/LConn1 -- Disp/RConn1
  Area B-T/RConn1 -- B-T/RConn1
  Reverse Direction/RConn1 -- Area P-B/LConn1 -- Area A-T/LConn1
  Area P-B/RConn1 -- B-P/RConn1
  Area A-T/RConn1 -- A-T/RConn1

== system ssc_hydraulic_lift/Load/Scissor/Actuator/Translational Simscape Intf ==
  Ideal Force Sensor : fl_lib/Mechanical/Mechanical Sensors/Ideal Force Sensor
  Ideal Translational Velocity Source : fl_lib/Mechanical/Mechanical Sources/Ideal Translational Velocity Source
  V : PMIOPort  Side=Right
  F : PMIOPort  Port=2  Side=Left
  R : PMIOPort  Port=3  Side=Right
  C : PMIOPort  Port=4  Side=Left
  connections:
  Ideal Translational Velocity Source/RConn1 -- V/RConn1
  F/RConn1 -- Ideal Force Sensor/RConn2
  Ideal Translational Velocity Source/LConn1 -- Ideal Force Sensor/RConn1
  Ideal Translational Velocity Source/RConn2 -- R/RConn1
  Ideal Force Sensor/LConn1 -- C/RConn1
